simulink model "sm_car"  (R2025a)
settings: Solver=ode23t  StartTime=0.0  StopTime=400  MaxStep=0.4  RelTol=1e-3  AbsTol=1e-3  EnableMultiTasking=on
PreLoadFcn:
  | % Due to usability issue in Repeating Sequence block
  | warning('off','Simulink:Masking:Invalid');
  | 
  | % Eliminate unnecessary warnings in inactive variants
  | % Warnings generated only if you click through inactive variant
  | warning('off','MATLAB:nonExistentField');
  | warning('off','Simulink:Parameters:BlkParamUndefined');
PostLoadFcn:
  | set_param([bdroot '/Vehicle'],'popup_trailer','Off')
  | warning('off','sm:sli:setup:compile:LocalSolverNotSupported')
  | %sm_car_config_maneuver(bdroot,'WOT Braking');
  | sm_car_config_vehicle(bdroot,'false');
  | sm_car_config_logging(bdroot);
InitFcn:
  | sm_car_config_camera;
  | Vehicle = sm_car_vehcfg_checkConfig(Vehicle);
  | sm_car_check_tire_model(bdroot);
StartFcn:
  | tic;
StopFcn:
  | Elapsed_Sim_Time = toc;
  | % disp(['Elapsed Sim Time = ' num2str(Elapsed_Sim_Time)]);
undefined symbols (not defined in the file): Axle1D, AxleIn, Camera, Control, Driver, Free, Init, Maneuver, Pedal, RaceFix, RaceSpin, Scene, ShaftL1, ShaftL2, ShaftR1, ShaftR2, Soft, Stiff, Visual, X, xy_data_car_side, Y, Z
libraries: sm_lib x1546, nesl_utility x528, fl_lib x480, SimscapeFluids_lib x61, sdl_lib x49, simulink x29, ee_lib x7, simulink_extras x6, Linkage_Systems x4, Tire_1x2x x4, AntiRollBar_Systems x2, Linkage_Decoupled x2
(part 48 of 79)

== system sm_car/Vehicle/Vehicle/Chassis/Spring/Decoupled/Spring A2 Roll/AirOilPiston/Sensor Gas Stiff T  ==
  PS-Simulink Converter10 : nesl_utility/PS-Simulink Converter  PhysicalDomain=network_engine_domain  SubClassName=ps_output  LeftPortType=input  RightPortType=output  PseudoPeriodic=off  Frequencies=[]  VectorFormat=inherit  Unit=degC  AffineConversion=on
  Temperature Sensor : fl_lib/Thermal/Thermal Sensors/Temperature Sensor  temperature_measure=foundation.enum.MeasurementReference.difference
  ThRef : fl_lib/Thermal/Thermal Elements/Thermal Reference
  A : PMIOPort  Side=Left
  T : Outport
  wires:
  PS-Simulink Converter10/1 -> T/1
  connections:
  ThRef/LConn1 -- Temperature Sensor/RConn1
  PS-Simulink Converter10/LConn1 -- Temperature Sensor/RConn2
  A/RConn1 -- Temperature Sensor/LConn1
